simulink model "E3_notAffectX1_3X1OnX2"  (R2024a)
settings: Solver=FixedStepAuto  StartTime=0.0  StopTime=10.0  FixedStep=0.01  RelTol=1e-3
libraries: simulink x1
settings Model: Creator=Sanagostar  LastModifiedBy=Sanagostar

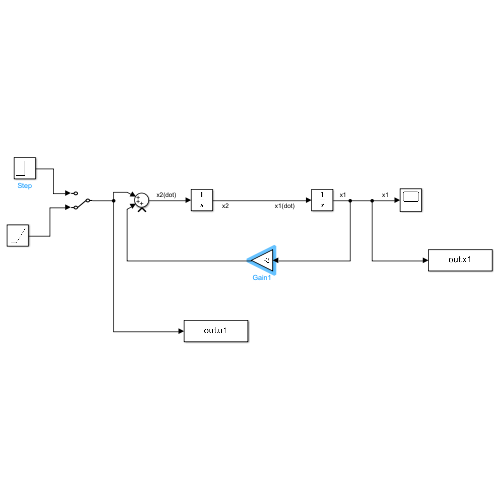
[thumbnail: Simulink's stored preview of the top-level diagram]
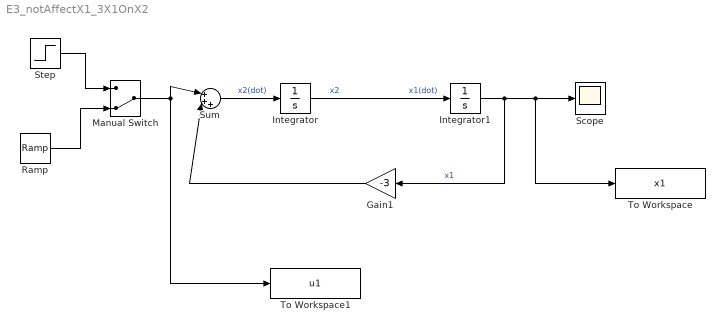
== system E3_notAffectX1_3X1OnX2 ==
  Gain1 : Gain  Gain=-3
  Integrator : Integrator
  Integrator1 : Integrator
  Manual Switch : ManualSwitch  CurrentSetting=0
  Ramp : simulink/Sources/Ramp  slope=1  start=0  InitialOutput=0
  Scope : Scope
  Step : Step  Time=0  SampleTime=0
  Sum : Sum  Inputs=|+++
  To Workspace : ToWorkspace  VariableName=x1  SaveFormat=Timeseries  SampleTime=-1
  To Workspace1 : ToWorkspace  VariableName=u1  SaveFormat=Timeseries  SampleTime=-1
  wires:
  Gain1/1 -> Sum/2
  Sum/1 -> Integrator/1  "x2(dot)"
  Integrator1/1 -> To Workspace/1, Scope/1, Gain1/1  "x1"
  Integrator/1 -> Integrator1/1  "x2                          x1(dot)"
  Step/1 -> Manual Switch/1
  Manual Switch/1 -> To Workspace1/1, Sum/1
  Ramp/1 -> Manual Switch/2
